simulink model "conveyor_belt_openloop"  (R2026a)
settings: Solver=ode4  StartTime=0  StopTime=20  FixedStep=0.01
PostLoadFcn:
  | mdlDir = fileparts(get_param('conveyor_belt_openloop', 'FileName'));
  | cadDir = fullfile(mdlDir, 'CAD');
  | addpath(cadDir);
  | prevDir = cd(cadDir);   % the copy in this folder wins over any other on the path
  | try
  |     convP = conveyor_belt_params();
  | catch paramsErr
  |     cd(prevDir); rethrow(paramsErr);
  | end
  | cd(prevDir);
  | missingFields = setdiff({'Ke', 'Tfric_Nm', 'bedFriction', 'beltDrag_N', 'beltTop_m', 'binFriction', 'contactOmega', 'contactZeta', 'controlPeriod_s', 'countsPerMotorRev', 'cycle_s', 'driverDrop_V', 'dropTimes_s', 'encWindow', 'frictionRate', 'g', 'gearEff', 'gearRatio', 'handOmega', 'handTime_s', 'itemFriction', 'itemMass_kg', 'itemSize_m', 'mmPerCount', 'motorR_ohm', 'rEff_m', 'restOffset_m', 'supplyV', 'vSlip', 'wSlip', 'xDrive_m', 'xDrop_m', 'xIdler_m', 'xReturn_m', 'zBinFloor_m', 'zCarry_m', 'zUnder_m', 'zWait_m'}, fieldnames(convP));
  | if ~isempty(missingFields)
  |     warning('Conveyor:params', '%s is older than this model (no %s). Replace it with the conveyor_belt_params.m that came with the model.', fullfile(cadDir, 'conveyor_belt_params.m'), strjoin(missingFields, ', '));
  | end
  | clear mdlDir cadDir prevDir missingFields
InitFcn:
  | mdlDir = fileparts(get_param('conveyor_belt_openloop', 'FileName'));
  | cadDir = fullfile(mdlDir, 'CAD');
  | addpath(cadDir);
  | prevDir = cd(cadDir);   % the copy in this folder wins over any other on the path
  | try
  |     convP = conveyor_belt_params();
  | catch paramsErr
  |     cd(prevDir); rethrow(paramsErr);
  | end
  | cd(prevDir);
  | missingFields = setdiff({'Ke', 'Tfric_Nm', 'bedFriction', 'beltDrag_N', 'beltTop_m', 'binFriction', 'contactOmega', 'contactZeta', 'controlPeriod_s', 'countsPerMotorRev', 'cycle_s', 'driverDrop_V', 'dropTimes_s', 'encWindow', 'frictionRate', 'g', 'gearEff', 'gearRatio', 'handOmega', 'handTime_s', 'itemFriction', 'itemMass_kg', 'itemSize_m', 'mmPerCount', 'motorR_ohm', 'rEff_m', 'restOffset_m', 'supplyV', 'vSlip', 'wSlip', 'xDrive_m', 'xDrop_m', 'xIdler_m', 'xReturn_m', 'zBinFloor_m', 'zCarry_m', 'zUnder_m', 'zWait_m'}, fieldnames(convP));
  | if isfield(convP, 'plaChain') && convP.plaChain ~= 0
  |     warning('Conveyor:belt', 'plaChain in conveyor_belt_params.m changed since this model was built: run build_conveyor_models so the 3-D parts match.');
  | end
  | if ~isempty(missingFields)
  |     error('Conveyor:params', '%s is older than this model (no %s). Replace it with the conveyor_belt_params.m that came with the model.', fullfile(cadDir, 'conveyor_belt_params.m'), strjoin(missingFields, ', '));
  | end
  | if ~strcmpi(pwd, mdlDir), cd(mdlDir); end   % STEP files are loaded as CAD/<part>.step
  | clear mdlDir cadDir prevDir missingFields
undefined symbols (not defined in the file or in its folder): X, Y, Z
libraries: sm_lib x73, nesl_utility x53, simulink x3, aerolibanimutils x1, slpidlib x1
(part 1 of 3)
settings Model: Creator=natha  LastModifiedBy=CadeP
settings SimscapeCC: SimscapeNominalValues="[{\"value\":\"1\",\"unit\":\"A\"},{\"value\":\"1\",\"unit\":\"bar\"},{\"value\":\"1\",\"unit\":\"cm^2\"},{\"value\":\"1\",\"unit\":\"cm^3/s\"},{\"value\":\"1\",\"unit\":\"kJ/kg\"},{\"value\":\"1\",\"unit\":\"kW\"},{\"value\":\"1\",\"unit\":\"l\"},{\"value\":\"1\",\"unit\":\"N\"},{\"value\":\"1\",\"unit\":\"N*m\"},{\"value\":\"1\",\"unit\":\"V\"}]"  SimscapeLogType=none  SimscapeLogDataHistory=5000.0

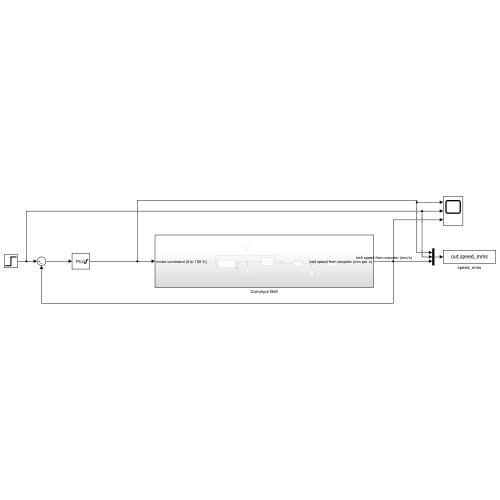
[thumbnail: Simulink's stored preview of the top-level diagram]
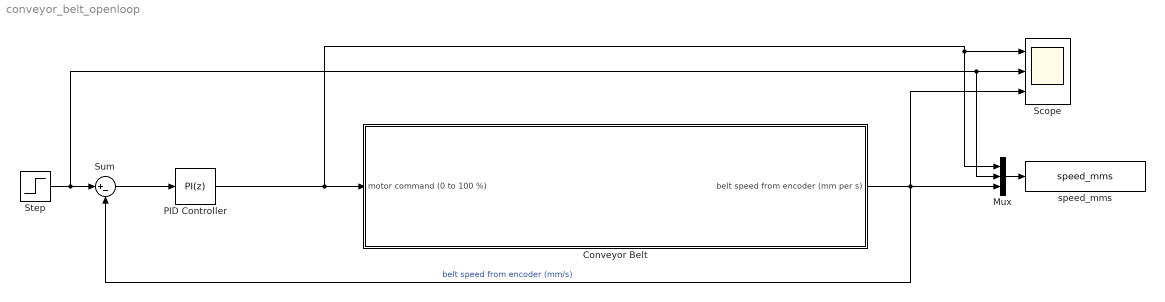
== system conveyor_belt_openloop ==
  Conveyor Belt : Subsystem
  Mux : Mux  Inputs=3
  PID Controller : slpidlib/PID Controller  Controller=PI  Form=Parallel  TimeDomain=Discrete-time  UseExternalTs=off  SampleTime=0.01  IntegratorMethod=Forward Euler  FilterMethod=Forward Euler  ControllerParametersSource=internal  P=0.0719  I=0.933  UseKiTs=off  D=0  UseExternalDerivativeSource=off  N=100  UseFilter=on  TunerSelectOption=Transfer Function Based (PID Tuner App)  InitialConditionSource=internal  InitialConditionForIntegrator=40  InitialConditionForFilter=0  DifferentiatorICPrevScaledInput=0  ExternalReset=none  TrackingMode=off  Kt=1  LimitOutput=on  SatLimitsSource=internal  UpperSaturationLimit=100  LowerSaturationLimit=25  LinearizeAsGain=on  AntiWindupMode=clamping  Kb=1  LimitIntegrator=off  UpperIntegratorSaturationLimit=inf  LowerIntegratorSaturationLimit=-inf  POutMin=[]  POutMax=[]  IOutMin=[]  IOutMax=[]  DOutMin=[]  DOutMax=[]  NOutMin=[]  NOutMax=[]  SumOutMin=[]  SumOutMax=[]  SaturationOutMin=[]  SaturationOutMax=[]  PParamMin=[]  PParamMax=[]  IParamMin=[]  IParamMax=[]  DParamMin=[]  DParamMax=[]  NParamMin=[]  NParamMax=[]  KbParamMin=[]  KbParamMax=[]  KtParamMin=[]  KtParamMax=[]  KbOutMin=[]  KbOutMax=[]  KtOutMin=[]  KtOutMax=[]  IntegratorOutMin=[]  IntegratorOutMax=[]  FilterOutMin=[]  FilterOutMax=[]  SumI1OutMin=[]  SumI1OutMax=[]  SumI2OutMin=[]  SumI2OutMax=[]  SumI3OutMin=[]  SumI3OutMax=[]  SumI4OutMin=[]  SumI4OutMax=[]  SumDOutMin=[]  SumDOutMax=[]  DifferentiatorOutMin=[]  DifferentiatorOutMax=[]  FilterDiffOutCoefMin=[]  FilterDiffOutCoefMax=[]  ReciprocalOutMin=[]  ReciprocalOutMax=[]  SumDenOutMin=[]  SumDenOutMax=[]  SumNumOutMin=[]  SumNumOutMax=[]  DivideOutMin=[]  DivideOutMax=[]  UdiffTsProdOutMin=[]  UdiffTsProdOutMax=[]  NTsProdOutMin=[]  NTsProdOutMax=[]  UintegralTsProdOutMin=[]  UintegralTsProdOutMax=[]  UngainTsProdOutMin=[]  UngainTsProdOutMax=[]  ClampingZeroOutDataTypeStr=Inherit: Inherit via back propagation  ClampingZeroOutMin=[]  ClampingZeroOutMax=[]  FilterDenConstantOutDataTypeStr=Inherit: Inherit via back propagation  FilterDenConstantOutMin=[]  FilterDenConstantOutMax=[]  PCopyOutDataTypeStr=Inherit: Inherit via back propagation  PCopyOutMin=[]  PCopyOutMax=[]  NCopyOutDataTypeStr=Inherit: Inherit via back propagation  NCopyOutMin=[]  NCopyOutMax=[]  IntegratorContinuousStateAttributes=''  IntegratorStateMustResolveToSignalObject=off  IntegratorRTWStateStorageClass=Auto  FilterContinuousStateAttributes=''  FilterStateMustResolveToSignalObject=off  FilterRTWStateStorageClass=Auto  ParallelPVariant=InternalParameters  IdealPVariant=Disabled  IVariant=InternalParameters  DVariant=Disabled  IntegratorVariant=Discrete  SatVariant=Enabled  AWVariant=DiscClampingParallel  PCopyVariant=Disabled  TRVariant=Disabled  FdbkBlocksVariant=Forward  IdealPFdbkVariant=Disabled  SatFdbkVariant=Disabled  DerivativeFilterVariant=Disabled  NVariant=Disabled  NCopyVariant=Disabled_SignalSpec  FilterICVariant=Disabled  IntegratorICVariant=InternalICs  ExternalResetVariant=Disabled  TRSumVariant=Passthrough  SumFdbkVariant=Disabled  SumVariant=Sum_PI  TsampFilterVariant=InternalTs  TsampNgainVariant=Passthrough  TsampIntegralVariant=Disabled_SignalSpec  ExternalSaturationOutDataTypeStr=Inherit: Same as second input  DerivativeSourceVariant=Disabled  PreIntVariant=InternalPreInt
  Scope : Scope  NumInputPorts=3
      settings: Title=motor command (% duty)  ActiveDisplayYMinimum=-122.04016461700802  ActiveDisplayYMaximum=1098.3614815530725
  Step : Step  Time=5  InitialValue=330  FinalValue=430  SampleTime=0
  Sum : Sum  Inputs=|+-
  speed_mms : ToWorkspace  VariableName=speed_mms  SaveFormat=Timeseries  SampleTime=-1
  wires:
  Conveyor Belt/1(belt speed from encoder (mm per s)) -> Sum/2, Mux/3, Scope/3  "belt speed from encoder (mm/s)"
  Mux/1 -> speed_mms/1
  PID Controller/1 -> Mux/1, Scope/1, Conveyor Belt/1(motor command (0 to 100 %))
  Step/1 -> Mux/2, Scope/2, Sum/1
  Sum/1 -> PID Controller/1

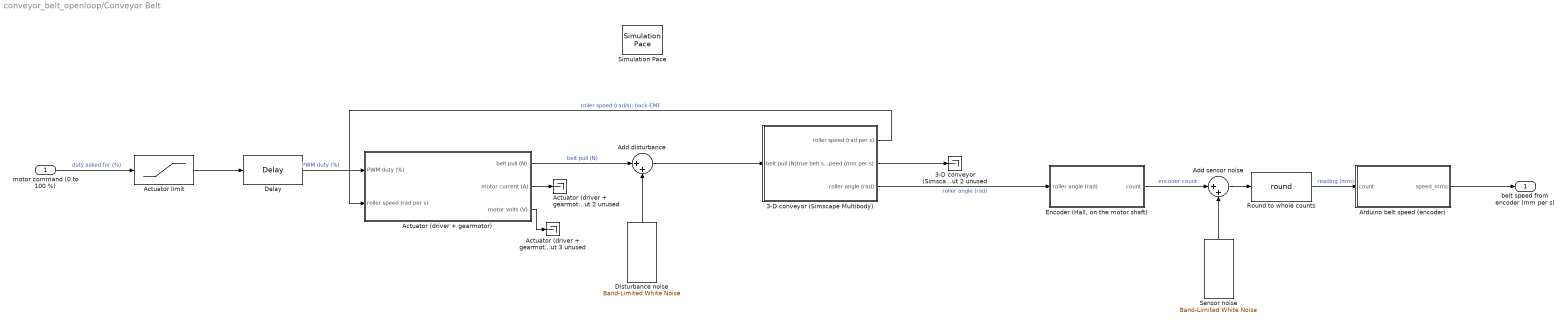
== system conveyor_belt_openloop/Conveyor Belt ==
  motor command (0 to 100 %) : Inport
  3-D conveyor (Simscape Multibody) : Subsystem
  3-D conveyor (Simscape Multibody) out 2 unused : Terminator
  Actuator (driver + gearmotor) : Subsystem
  Actuator (driver + gearmotor) out 2 unused : Terminator
  Actuator (driver + gearmotor) out 3 unused : Terminator
  Actuator limit : Saturate  UpperLimit=100  LowerLimit=0
  Add disturbance : Sum  Inputs=|++
  Add sensor noise : Sum  Inputs=|++
  Arduino belt speed (encoder) : MATLAB Function  TreatAsAtomicUnit=on
  Delay : TransportDelay  DelayTime=convP.delayBlock_s
  Disturbance noise : simulink/Sources/Band-Limited White Noise  Cov=convP.dragNoiseCov  Ts=convP.dragNoiseTs_s  seed=convP.noiseSeed + 1
  "Encoder (Hall, on the motor shaft)" : Subsystem
  Round to whole counts : Rounding  Operator=round
  Sensor noise : simulink/Sources/Band-Limited White Noise  Cov=0  Ts=0.01  seed=convP.noiseSeed
  Simulation Pace : aerolibanimutils/Simulation Pace  SimulationPace=1  SleepMode=Auto  OutputPaceError=off  SampleTime=-1
  belt speed from encoder (mm per s) : Outport
  wires:
  motor command (0 to 100 %)/1 -> Actuator limit/1  "duty asked for (%)"
  Actuator limit/1 -> Delay/1
  Delay/1 -> Actuator (driver + gearmotor)/1(PWM duty (%))  "PWM duty (%)"
  Actuator (driver + gearmotor)/1(belt pull (N)) -> Add disturbance/1  "belt pull (N)"
  Disturbance noise/1 -> Add disturbance/2
  Add disturbance/1 -> 3-D conveyor (Simscape Multibody)/1(belt pull (N))
  3-D conveyor (Simscape Multibody)/1(roller speed (rad per s)) -> Actuator (driver + gearmotor)/2(roller speed (rad per s))  "roller speed (rad/s): back-EMF"
  3-D conveyor (Simscape Multibody)/3(roller angle (rad)) -> "Encoder (Hall, on the motor shaft)"/1(roller angle (rad))  "roller angle (rad)"
  "Encoder (Hall, on the motor shaft)"/1(count) -> Add sensor noise/1  "encoder count"
  3-D conveyor (Simscape Multibody)/2(true belt speed (mm per s)) -> 3-D conveyor (Simscape Multibody) out 2 unused/1
  Actuator (driver + gearmotor)/2(motor current (A)) -> Actuator (driver + gearmotor) out 2 unused/1
  Actuator (driver + gearmotor)/3(motor volts (V)) -> Actuator (driver + gearmotor) out 3 unused/1
  Arduino belt speed (encoder)/1(speed_mms) -> belt speed from encoder (mm per s)/1
  Sensor noise/1 -> Add sensor noise/2
  Add sensor noise/1 -> Round to whole counts/1
  Round to whole counts/1 -> Arduino belt speed (encoder)/1(count)  "reading (mm)"

== system conveyor_belt_openloop/Conveyor Belt/3-D conveyor (Simscape Multibody) ==
  belt pull (N) : Inport
  Belt and item contact : MATLAB Function  TreatAsAtomicUnit=on
  Clock : Clock
  Drive roller : Subsystem
  Frame (fixed parts) : Subsystem
  Idler (follows the drive roller) : Subsystem
  Items : Subsystem
  Mechanism (gravity -Z) : sm_lib/Utilities/Mechanism Configuration  UniformGravity=Constant  GravityVector=[0 0 -9.80665]  GravityVectorUnits=m/s^2  LinearizationDelta=0.001  JointModeTransitionNonlinearIterations=2
  Net belt force : Sum  Inputs=|+-
  Solver : nesl_utility/Solver Configuration  PhysicalDomain=network_engine_domain  SubClassName=solver  LeftPortType=input  RightPortType=generic  Tones=[]  Harmonics=[]  SimulateNoise=off  Profile=off  UseLocalSampling=off  EnableSwitchedLinearOptims=on  FrequencyDomain=off  UseCCode=off  RelTol=0.001  AbsTol=0.001  MinStep=1e-09  ToWorkspace=off  RevertToSquareIcSolve=off  NumHomotopyIterations=100  PhasorMode=off  PhasorModeNumHarmonics=1  ConsistencySolver=NEWTON_XTOL_AFTER_FTOL  CanonicalOrdering=UNORDERED  OptimizeIntermediates=UNOPTIMIZED  IndexReductionMethod=DerivativeReplacement  DoDC=off  ResidualTolerance=1e-09  ConsistencyTolSource=GLOBAL  ConsistencyAbsTol=0.001  ConsistencyRelTol=0.001  ConsistencyTolFactor=0.001  UseLocalSolver=off  LocalSolverChoice=NE_BACKWARD_EULER_ADVANCER  ResolveIndetEquations=on  FunctionEvalNumThread=1  LocalSolverSampleTime=0.001  DoFixedCost=off  MaxNonlinIter=3  MaxModeIter=2  ComputeImpulses=off  ImpulseIterations=2  LinearAlgebra=auto  LinearAlgebraNumThread=0  EquationFormulation=NE_TIME_EF  DelaysMemoryBudget=1024  AutomaticFiltering=on  FilteringTimeConstant=0.001  PartitionStorageMethod=AS_NEEDED  PartitionMemoryBudget=1024  PartitionMethod=ROBUST  MultibodyUseLocalSolver=off  MultibodyLocalSolverChoice=ODE1  MultibodyLocalSolverSampleTime=0.001
  World : sm_lib/Frames and Transforms/World Frame
  belt speed (m per s) : Gain  Gain=convP.rEff_m
  times roller radius : Gain  Gain=convP.rEff_m
  to mm per s : Gain  Gain=1000
  roller speed (rad per s) : Outport
  true belt speed (mm per s) : Outport  Port=2
  roller angle (rad) : Outport  Port=3
  wires:
  belt pull (N)/1 -> Net belt force/1
  Belt and item contact/3(Fload) -> Net belt force/2  "load from items + bed drag (N)"
  Net belt force/1 -> times roller radius/1
  times roller radius/1 -> Drive roller/1(torque (N m))  "torque (N m)"
  Drive roller/1(angle (rad)) -> Idler (follows the drive roller)/1(drive roller angle (rad)), roller angle (rad)/1
  Drive roller/2(speed (rad per s)) -> belt speed (m per s)/1, roller speed (rad per s)/1
  belt speed (m per s)/1 -> Belt and item contact/5(vBelt), to mm per s/1
  to mm per s/1 -> true belt speed (mm per s)/1
  Clock/1 -> Belt and item contact/6(tNow)
  Items/1(x from drop point (m)) -> Belt and item contact/1(px)
  Items/2(z from drop point (m)) -> Belt and item contact/2(pz)
  Items/3(vx (m per s)) -> Belt and item contact/3(vx)
  Items/4(vz (m per s)) -> Belt and item contact/4(vz)
  Belt and item contact/1(Fx) -> Items/1(Fx (N))
  Belt and item contact/2(Fz) -> Items/2(Fz (N))
  connections:
  Solver/RConn1 -- World/RConn1 -- Items/LConn1 -- Drive roller/LConn1 -- Idler (follows the drive roller)/LConn1 -- Frame (fixed parts)/LConn1 -- Mechanism (gravity -Z)/RConn1

== system conveyor_belt_openloop/Conveyor Belt/Actuator (driver + gearmotor) ==
  PWM duty (%) : Inport
  roller speed (rad per s) : Inport  Port=2
  DC motor and gearbox : MATLAB Function  TreatAsAtomicUnit=on
  duty to volts : Gain  Gain=convP.supplyV/100
  belt pull (N) : Outport
  motor current (A) : Outport  Port=2
  motor volts (V) : Outport  Port=3
  wires:
  PWM duty (%)/1 -> duty to volts/1
  duty to volts/1 -> DC motor and gearbox/1(Vcmd)
  roller speed (rad per s)/1 -> DC motor and gearbox/2(wRoller)
  DC motor and gearbox/1(Fpull) -> belt pull (N)/1
  DC motor and gearbox/2(current) -> motor current (A)/1
  DC motor and gearbox/3(Vmotor) -> motor volts (V)/1

== system conveyor_belt_openloop/Conveyor Belt/Encoder (Hall, on the motor shaft) ==
  roller angle (rad) : Inport
  Edge jitter : simulink/Sources/Band-Limited White Noise  Cov=convP.encNoiseCov  Ts=convP.controlPeriod_s  seed=convP.noiseSeed + 2
  Hall encoder count : MATLAB Function  TreatAsAtomicUnit=on
  Read the count every 10 ms : ZeroOrderHold  SampleTime=convP.controlPeriod_s
  count : Outport
  wires:
  roller angle (rad)/1 -> Read the count every 10 ms/1
  Read the count every 10 ms/1 -> Hall encoder count/1(angle_rad)
  Edge jitter/1 -> Hall encoder count/2(jitter_counts)
  Hall encoder count/1(count) -> count/1

== system conveyor_belt_openloop/Conveyor Belt/3-D conveyor (Simscape Multibody)/Drive roller ==
  torque (N m) : Inport
  Drive axis : sm_lib/Frames and Transforms/Rigid Transform  RotationMethod=StandardAxis  FollAlignAxisA=+X  BaseAlignAxisA=+Y  FollAlignAxisB=+Y  BaseAlignAxisB=+Z  RotationStandardAxis=+X  RotationAngle=-90  RotationAngleUnits=deg  RotationArbitraryAxis=[0 0 1]  RotationSequenceAxes=FollowerAxes  RotationSequence=XYX  RotationSequenceAngles=[0 0 0]  RotationSequenceAnglesUnits=deg  RotationMatrix=[1 0 0;0 1 0;0 0 1]  Quaternion=[1 0 0 0]  TranslationMethod=Cartesian  TranslationCartesianOffset=[convP.xDrive_m 0 convP.zAxis_m]  TranslationCartesianOffsetUnits=m  TranslationStandardAxis=+Z  TranslationStandardOffset=0  TranslationStandardOffsetUnits=m  TranslationROffset=0  TranslationROffsetUnits=m  TranslationThetaOffset=0  TranslationThetaOffsetUnits=deg  TranslationZOffset=0  TranslationZOffsetUnits=m
  Drive roller bearings : sm_lib/Joints/Revolute Joint  JointMode=Normal  CompositeWrenchDir=FollowerOnBase  CompositeWrenchFrame=BaseFrame  SenseConstraintForce=off  SenseConstraintTorque=off  SenseTotalForce=off  SenseTotalTorque=off  PositionTargetSpecify=off  PositionTargetPriority=High  PositionTargetValue=0  PositionTargetValueUnits=deg  VelocityTargetSpecify=off  VelocityTargetPriority=High  VelocityTargetValue=0  VelocityTargetValueUnits=deg/s  EquilibriumPosition=0  EquilibriumPositionUnits=deg  SpringStiffness=0  SpringStiffnessUnits=N*m/deg  DampingCoefficient=0  DampingCoefficientUnits=N*m/(deg/s)  LowerLimitSpecify=off  LowerLimitBound=-90  LowerLimitBoundUnits=deg  LowerLimitStiffness=1e4  LowerLimitStiffnessUnits=N*m/deg  LowerLimitDamping=10  LowerLimitDampingUnits=N*m/(deg/s)  LowerLimitTransitionRegionWidth=0.1  LowerLimitTransitionRegionWidthUnits=deg  UpperLimitSpecify=off  UpperLimitBound=90  UpperLimitBoundUnits=deg  UpperLimitStiffness=1e4  UpperLimitStiffnessUnits=N*m/deg  UpperLimitDamping=10  UpperLimitDampingUnits=N*m/(deg/s)  UpperLimitTransitionRegionWidth=0.1  UpperLimitTransitionRegionWidthUnits=deg  TorqueActuationMode=InputTorque  MotionActuationMode=ComputedMotion  SensePosition=on  SenseVelocity=on  SenseAcceleration=off  SenseTorqueForce=off  SenseLowerLimitTorqueForce=off  SenseUpperLimitTorqueForce=off
  Motor rotor (reflected inertia) : sm_lib/Body Elements/Inertia  InertiaType=Custom  Mass=0.01  MassUnits=kg  CenterOfMass=[0 0 0]  CenterOfMassUnits=m  MomentsOfInertia=[1 1 1]*convP.J_drive  MomentsOfInertiaUnits=kg*m^2  ProductsOfInertia=[0 0 0]  ProductsOfInertiaUnits=kg*m^2  GraphicType=Marker  MarkerShape=Inertia  MarkerSize=20  GraphicVisPropType=SimpleVisualProperties  GraphicDiffuseColor=[0.5 0.5 0.5]  GraphicOpacity=1  GraphicSpecularColor=[0.5 0.5 0.5 1.0]  GraphicAmbientColor=[0.15 0.15 0.15 1.0]  GraphicEmissiveColor=[0.0 0.0 0.0 1.0]  GraphicShininess=75
  Other half faces the other way : sm_lib/Frames and Transforms/Rigid Transform  RotationMethod=StandardAxis  FollAlignAxisA=+X  BaseAlignAxisA=+Y  FollAlignAxisB=+Y  BaseAlignAxisB=+Z  RotationStandardAxis=+X  RotationAngle=180  RotationAngleUnits=deg  RotationArbitraryAxis=[0 0 1]  RotationSequenceAxes=FollowerAxes  RotationSequence=XYX  RotationSequenceAngles=[0 0 0]  RotationSequenceAnglesUnits=deg  RotationMatrix=[1 0 0;0 1 0;0 0 1]  Quaternion=[1 0 0 0]  TranslationMethod=None  TranslationCartesianOffset=[0 0 0]  TranslationCartesianOffsetUnits=m  TranslationStandardAxis=+Z  TranslationStandardOffset=0  TranslationStandardOffsetUnits=m  TranslationROffset=0  TranslationROffsetUnits=m  TranslationThetaOffset=0  TranslationThetaOffsetUnits=deg  TranslationZOffset=0  TranslationZOffsetUnits=m
  Roller half (drive end) : sm_lib/Body Elements/File Solid  ExtGeomFileName=CAD/roller_half_drive.step  UnitType=FromFile  ExtGeomFileUnits=m  StepReaderType=HEX  ExportConvexHullGeometry=off  InertiaType=CalculateFromGeometry  BasedOnType=Density  Density=convP.printDensity_kgm3  DensityUnits=kg/m^3  Mass=1  MassUnits=kg  CenterOfMass=[0 0 0]  CenterOfMassUnits=m  MomentsOfInertia=[1 1 1]  MomentsOfInertiaUnits=kg*m^2  ProductsOfInertia=[0 0 0]  ProductsOfInertiaUnits=kg*m^2  GraphicType=FromGeometry  MarkerShape=Sphere  MarkerSize=10  GraphicVisPropType=SimpleVisualProperties  GraphicDiffuseColor=[0.92 0.92 0.92]  GraphicOpacity=1  GraphicSpecularColor=[0.5 0.5 0.5 1.0]  GraphicAmbientColor=[0.15 0.15 0.15 1.0]  GraphicEmissiveColor=[0.0 0.0 0.0 1.0]  GraphicShininess=75  DoExposeReferenceFrame=on  SerializedFrames=<Frames/>
  Roller half (plain end) : sm_lib/Body Elements/File Solid  ExtGeomFileName=CAD/roller_half_plain.step  UnitType=FromFile  ExtGeomFileUnits=m  StepReaderType=HEX  ExportConvexHullGeometry=off  InertiaType=CalculateFromGeometry  BasedOnType=Density  Density=convP.printDensity_kgm3  DensityUnits=kg/m^3  Mass=1  MassUnits=kg  CenterOfMass=[0 0 0]  CenterOfMassUnits=m  MomentsOfInertia=[1 1 1]  MomentsOfInertiaUnits=kg*m^2  ProductsOfInertia=[0 0 0]  ProductsOfInertiaUnits=kg*m^2  GraphicType=FromGeometry  MarkerShape=Sphere  MarkerSize=10  GraphicVisPropType=SimpleVisualProperties  GraphicDiffuseColor=[0.92 0.92 0.92]  GraphicOpacity=1  GraphicSpecularColor=[0.5 0.5 0.5 1.0]  GraphicAmbientColor=[0.15 0.15 0.15 1.0]  GraphicEmissiveColor=[0.0 0.0 0.0 1.0]  GraphicShininess=75  DoExposeReferenceFrame=on  SerializedFrames=<Frames/>
  angle out : nesl_utility/PS-Simulink Converter  PhysicalDomain=network_engine_domain  SubClassName=ps_output  LeftPortType=input  RightPortType=output  PseudoPeriodic=off  Frequencies=[]  VectorFormat=inherit  Unit=rad  AffineConversion=off
  speed out : nesl_utility/PS-Simulink Converter  PhysicalDomain=network_engine_domain  SubClassName=ps_output  LeftPortType=input  RightPortType=output  PseudoPeriodic=off  Frequencies=[]  VectorFormat=inherit  Unit=rad/s  AffineConversion=off
  torque to physical : nesl_utility/Simulink-PS Converter  PhysicalDomain=network_engine_domain  SubClassName=ps_input  LeftPortType=input  RightPortType=output  PseudoPeriodic=off  Frequencies=[]  NoiseDistribution=none  NoiseParameters=[]  Unit=N*m  AffineConversion=off  FilteringAndDerivatives=provide  SimscapeFilterOrder=1  InputFilterTimeConstant=0.001  UdotUserProvided=0
  W : PMIOPort  Side=Left
  angle (rad) : Outport
  speed (rad per s) : Outport  Port=2
  wires:
  torque (N m)/1 -> torque to physical/1
  angle out/1 -> angle (rad)/1
  speed out/1 -> speed (rad per s)/1
  connections:
  W/RConn1 -- Drive axis/LConn1
  Drive axis/RConn1 -- Drive roller bearings/LConn1
  torque to physical/RConn1 -- Drive roller bearings/LConn2
  Roller half (drive end)/RConn1 -- Drive roller bearings/RConn1 -- Other half faces the other way/LConn1 -- Motor rotor (reflected inertia)/RConn1
  Other half faces the other way/RConn1 -- Roller half (plain end)/RConn1
  Drive roller bearings/RConn2 -- angle out/LConn1
  Drive roller bearings/RConn3 -- speed out/LConn1

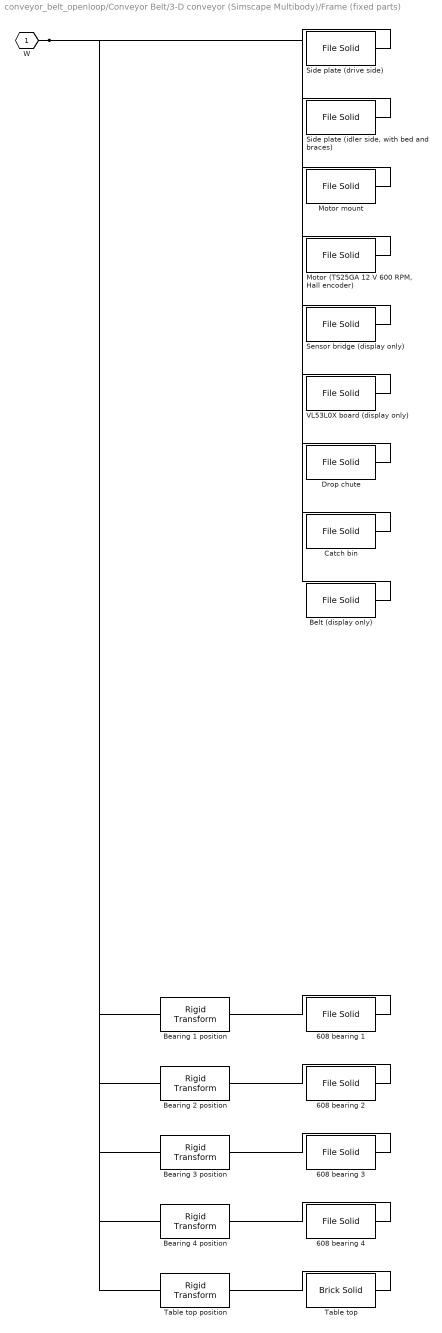
== system conveyor_belt_openloop/Conveyor Belt/3-D conveyor (Simscape Multibody)/Frame (fixed parts) ==
  608 bearing {1..4} (4 alike) : sm_lib/Body Elements/File Solid  ExtGeomFileName=CAD/bearing_608.step  UnitType=FromFile  ExtGeomFileUnits=m  StepReaderType=HEX  ExportConvexHullGeometry=off  InertiaType=CalculateFromGeometry  BasedOnType=Density  Density=convP.printDensity_kgm3  DensityUnits=kg/m^3  Mass=1  MassUnits=kg  CenterOfMass=[0 0 0]  CenterOfMassUnits=m  MomentsOfInertia=[1 1 1]  MomentsOfInertiaUnits=kg*m^2  ProductsOfInertia=[0 0 0]  ProductsOfInertiaUnits=kg*m^2  GraphicType=FromGeometry  MarkerShape=Sphere  MarkerSize=10  GraphicVisPropType=SimpleVisualProperties  GraphicDiffuseColor=[0.6 0.6 0.65]  GraphicOpacity=1  GraphicSpecularColor=[0.5 0.5 0.5 1.0]  GraphicAmbientColor=[0.15 0.15 0.15 1.0]  GraphicEmissiveColor=[0.0 0.0 0.0 1.0]  GraphicShininess=75  DoExposeReferenceFrame=on  SerializedFrames=<Frames/>
  Bearing 1 position : sm_lib/Frames and Transforms/Rigid Transform  RotationMethod=StandardAxis  FollAlignAxisA=+X  BaseAlignAxisA=+Y  FollAlignAxisB=+Y  BaseAlignAxisB=+Z  RotationStandardAxis=+X  RotationAngle=-90  RotationAngleUnits=deg  RotationArbitraryAxis=[0 0 1]  RotationSequenceAxes=FollowerAxes  RotationSequence=XYX  RotationSequenceAngles=[0 0 0]  RotationSequenceAnglesUnits=deg  RotationMatrix=[1 0 0;0 1 0;0 0 1]  Quaternion=[1 0 0 0]  TranslationMethod=Cartesian  TranslationCartesianOffset=[convP.xDrive_m convP.bearingY_m(1) convP.zAxis_m]  TranslationCartesianOffsetUnits=m  TranslationStandardAxis=+Z  TranslationStandardOffset=0  TranslationStandardOffsetUnits=m  TranslationROffset=0  TranslationROffsetUnits=m  TranslationThetaOffset=0  TranslationThetaOffsetUnits=deg  TranslationZOffset=0  TranslationZOffsetUnits=m
  Bearing 2 position : sm_lib/Frames and Transforms/Rigid Transform  RotationMethod=StandardAxis  FollAlignAxisA=+X  BaseAlignAxisA=+Y  FollAlignAxisB=+Y  BaseAlignAxisB=+Z  RotationStandardAxis=+X  RotationAngle=-90  RotationAngleUnits=deg  RotationArbitraryAxis=[0 0 1]  RotationSequenceAxes=FollowerAxes  RotationSequence=XYX  RotationSequenceAngles=[0 0 0]  RotationSequenceAnglesUnits=deg  RotationMatrix=[1 0 0;0 1 0;0 0 1]  Quaternion=[1 0 0 0]  TranslationMethod=Cartesian  TranslationCartesianOffset=[convP.xDrive_m convP.bearingY_m(2) convP.zAxis_m]  TranslationCartesianOffsetUnits=m  TranslationStandardAxis=+Z  TranslationStandardOffset=0  TranslationStandardOffsetUnits=m  TranslationROffset=0  TranslationROffsetUnits=m  TranslationThetaOffset=0  TranslationThetaOffsetUnits=deg  TranslationZOffset=0  TranslationZOffsetUnits=m
  Bearing 3 position : sm_lib/Frames and Transforms/Rigid Transform  RotationMethod=StandardAxis  FollAlignAxisA=+X  BaseAlignAxisA=+Y  FollAlignAxisB=+Y  BaseAlignAxisB=+Z  RotationStandardAxis=+X  RotationAngle=-90  RotationAngleUnits=deg  RotationArbitraryAxis=[0 0 1]  RotationSequenceAxes=FollowerAxes  RotationSequence=XYX  RotationSequenceAngles=[0 0 0]  RotationSequenceAnglesUnits=deg  RotationMatrix=[1 0 0;0 1 0;0 0 1]  Quaternion=[1 0 0 0]  TranslationMethod=Cartesian  TranslationCartesianOffset=[convP.xIdler_m convP.bearingY_m(1) convP.zAxis_m]  TranslationCartesianOffsetUnits=m  TranslationStandardAxis=+Z  TranslationStandardOffset=0  TranslationStandardOffsetUnits=m  TranslationROffset=0  TranslationROffsetUnits=m  TranslationThetaOffset=0  TranslationThetaOffsetUnits=deg  TranslationZOffset=0  TranslationZOffsetUnits=m
  Bearing 4 position : sm_lib/Frames and Transforms/Rigid Transform  RotationMethod=StandardAxis  FollAlignAxisA=+X  BaseAlignAxisA=+Y  FollAlignAxisB=+Y  BaseAlignAxisB=+Z  RotationStandardAxis=+X  RotationAngle=-90  RotationAngleUnits=deg  RotationArbitraryAxis=[0 0 1]  RotationSequenceAxes=FollowerAxes  RotationSequence=XYX  RotationSequenceAngles=[0 0 0]  RotationSequenceAnglesUnits=deg  RotationMatrix=[1 0 0;0 1 0;0 0 1]  Quaternion=[1 0 0 0]  TranslationMethod=Cartesian  TranslationCartesianOffset=[convP.xIdler_m convP.bearingY_m(2) convP.zAxis_m]  TranslationCartesianOffsetUnits=m  TranslationStandardAxis=+Z  TranslationStandardOffset=0  TranslationStandardOffsetUnits=m  TranslationROffset=0  TranslationROffsetUnits=m  TranslationThetaOffset=0  TranslationThetaOffsetUnits=deg  TranslationZOffset=0  TranslationZOffsetUnits=m
  Belt (display only) : sm_lib/Body Elements/File Solid  ExtGeomFileName=CAD/belt_installed_display.step  UnitType=FromFile  ExtGeomFileUnits=m  StepReaderType=HEX  ExportConvexHullGeometry=off  InertiaType=CalculateFromGeometry  BasedOnType=Density  Density=convP.printDensity_kgm3  DensityUnits=kg/m^3  Mass=1  MassUnits=kg  CenterOfMass=[0 0 0]  CenterOfMassUnits=m  MomentsOfInertia=[1 1 1]  MomentsOfInertiaUnits=kg*m^2  ProductsOfInertia=[0 0 0]  ProductsOfInertiaUnits=kg*m^2  GraphicType=FromGeometry  MarkerShape=Sphere  MarkerSize=10  GraphicVisPropType=SimpleVisualProperties  GraphicDiffuseColor=[0.1 0.1 0.1]  GraphicOpacity=1  GraphicSpecularColor=[0.5 0.5 0.5 1.0]  GraphicAmbientColor=[0.15 0.15 0.15 1.0]  GraphicEmissiveColor=[0.0 0.0 0.0 1.0]  GraphicShininess=75  DoExposeReferenceFrame=on  SerializedFrames=<Frames/>
  Catch bin : sm_lib/Body Elements/File Solid  ExtGeomFileName=CAD/catch_bin.step  UnitType=FromFile  ExtGeomFileUnits=m  StepReaderType=HEX  ExportConvexHullGeometry=off  InertiaType=CalculateFromGeometry  BasedOnType=Density  Density=convP.printDensity_kgm3  DensityUnits=kg/m^3  Mass=1  MassUnits=kg  CenterOfMass=[0 0 0]  CenterOfMassUnits=m  MomentsOfInertia=[1 1 1]  MomentsOfInertiaUnits=kg*m^2  ProductsOfInertia=[0 0 0]  ProductsOfInertiaUnits=kg*m^2  GraphicType=FromGeometry  MarkerShape=Sphere  MarkerSize=10  GraphicVisPropType=SimpleVisualProperties  GraphicDiffuseColor=[0.45 0.45 0.45]  GraphicOpacity=1  GraphicSpecularColor=[0.5 0.5 0.5 1.0]  GraphicAmbientColor=[0.15 0.15 0.15 1.0]  GraphicEmissiveColor=[0.0 0.0 0.0 1.0]  GraphicShininess=75  DoExposeReferenceFrame=on  SerializedFrames=<Frames/>
  Drop chute : sm_lib/Body Elements/File Solid  ExtGeomFileName=CAD/drop_chute.step  UnitType=FromFile  ExtGeomFileUnits=m  StepReaderType=HEX  ExportConvexHullGeometry=off  InertiaType=CalculateFromGeometry  BasedOnType=Density  Density=convP.printDensity_kgm3  DensityUnits=kg/m^3  Mass=1  MassUnits=kg  CenterOfMass=[0 0 0]  CenterOfMassUnits=m  MomentsOfInertia=[1 1 1]  MomentsOfInertiaUnits=kg*m^2  ProductsOfInertia=[0 0 0]  ProductsOfInertiaUnits=kg*m^2  GraphicType=FromGeometry  MarkerShape=Sphere  MarkerSize=10  GraphicVisPropType=SimpleVisualProperties  GraphicDiffuseColor=[0.15 0.65 0.35]  GraphicOpacity=1  GraphicSpecularColor=[0.5 0.5 0.5 1.0]  GraphicAmbientColor=[0.15 0.15 0.15 1.0]  GraphicEmissiveColor=[0.0 0.0 0.0 1.0]  GraphicShininess=75  DoExposeReferenceFrame=on  SerializedFrames=<Frames/>
  "Motor (TS25GA 12 V 600 RPM, Hall encoder)" : sm_lib/Body Elements/File Solid  ExtGeomFileName=CAD/motor_ts25ga_12v.step  UnitType=FromFile  ExtGeomFileUnits=m  StepReaderType=HEX  ExportConvexHullGeometry=off  InertiaType=CalculateFromGeometry  BasedOnType=Density  Density=convP.printDensity_kgm3  DensityUnits=kg/m^3  Mass=1  MassUnits=kg  CenterOfMass=[0 0 0]  CenterOfMassUnits=m  MomentsOfInertia=[1 1 1]  MomentsOfInertiaUnits=kg*m^2  ProductsOfInertia=[0 0 0]  ProductsOfInertiaUnits=kg*m^2  GraphicType=FromGeometry  MarkerShape=Sphere  MarkerSize=10  GraphicVisPropType=SimpleVisualProperties  GraphicDiffuseColor=[0.8 0.8 0.85]  GraphicOpacity=1  GraphicSpecularColor=[0.5 0.5 0.5 1.0]  GraphicAmbientColor=[0.15 0.15 0.15 1.0]  GraphicEmissiveColor=[0.0 0.0 0.0 1.0]  GraphicShininess=75  DoExposeReferenceFrame=on  SerializedFrames=<Frames/>
  Motor mount : sm_lib/Body Elements/File Solid  ExtGeomFileName=CAD/motor_mount.step  UnitType=FromFile  ExtGeomFileUnits=m  StepReaderType=HEX  ExportConvexHullGeometry=off  InertiaType=CalculateFromGeometry  BasedOnType=Density  Density=convP.printDensity_kgm3  DensityUnits=kg/m^3  Mass=1  MassUnits=kg  CenterOfMass=[0 0 0]  CenterOfMassUnits=m  MomentsOfInertia=[1 1 1]  MomentsOfInertiaUnits=kg*m^2  ProductsOfInertia=[0 0 0]  ProductsOfInertiaUnits=kg*m^2  GraphicType=FromGeometry  MarkerShape=Sphere  MarkerSize=10  GraphicVisPropType=SimpleVisualProperties  GraphicDiffuseColor=[0.25 0.75 0.85]  GraphicOpacity=1  GraphicSpecularColor=[0.5 0.5 0.5 1.0]  GraphicAmbientColor=[0.15 0.15 0.15 1.0]  GraphicEmissiveColor=[0.0 0.0 0.0 1.0]  GraphicShininess=75  DoExposeReferenceFrame=on  SerializedFrames=<Frames/>
  Sensor bridge (display only) : sm_lib/Body Elements/File Solid  ExtGeomFileName=CAD/sensor_bridge.step  UnitType=FromFile  ExtGeomFileUnits=m  StepReaderType=HEX  ExportConvexHullGeometry=off  InertiaType=CalculateFromGeometry  BasedOnType=Density  Density=convP.printDensity_kgm3  DensityUnits=kg/m^3  Mass=1  MassUnits=kg  CenterOfMass=[0 0 0]  CenterOfMassUnits=m  MomentsOfInertia=[1 1 1]  MomentsOfInertiaUnits=kg*m^2  ProductsOfInertia=[0 0 0]  ProductsOfInertiaUnits=kg*m^2  GraphicType=FromGeometry  MarkerShape=Sphere  MarkerSize=10  GraphicVisPropType=SimpleVisualProperties  GraphicDiffuseColor=[0.15 0.65 0.35]  GraphicOpacity=1  GraphicSpecularColor=[0.5 0.5 0.5 1.0]  GraphicAmbientColor=[0.15 0.15 0.15 1.0]  GraphicEmissiveColor=[0.0 0.0 0.0 1.0]  GraphicShininess=75  DoExposeReferenceFrame=on  SerializedFrames=<Frames/>
  Side plate (drive side) : sm_lib/Body Elements/File Solid  ExtGeomFileName=CAD/side_plate_drive.step  UnitType=FromFile  ExtGeomFileUnits=m  StepReaderType=HEX  ExportConvexHullGeometry=off  InertiaType=CalculateFromGeometry  BasedOnType=Density  Density=convP.printDensity_kgm3  DensityUnits=kg/m^3  Mass=1  MassUnits=kg  CenterOfMass=[0 0 0]  CenterOfMassUnits=m  MomentsOfInertia=[1 1 1]  MomentsOfInertiaUnits=kg*m^2  ProductsOfInertia=[0 0 0]  ProductsOfInertiaUnits=kg*m^2  GraphicType=FromGeometry  MarkerShape=Sphere  MarkerSize=10  GraphicVisPropType=SimpleVisualProperties  GraphicDiffuseColor=[0.25 0.45 0.85]  GraphicOpacity=1  GraphicSpecularColor=[0.5 0.5 0.5 1.0]  GraphicAmbientColor=[0.15 0.15 0.15 1.0]  GraphicEmissiveColor=[0.0 0.0 0.0 1.0]  GraphicShininess=75  DoExposeReferenceFrame=on  SerializedFrames=<Frames/>
  "Side plate (idler side, with bed and braces)" : sm_lib/Body Elements/File Solid  ExtGeomFileName=CAD/side_plate_idler.step  UnitType=FromFile  ExtGeomFileUnits=m  StepReaderType=HEX  ExportConvexHullGeometry=off  InertiaType=CalculateFromGeometry  BasedOnType=Density  Density=convP.printDensity_kgm3  DensityUnits=kg/m^3  Mass=1  MassUnits=kg  CenterOfMass=[0 0 0]  CenterOfMassUnits=m  MomentsOfInertia=[1 1 1]  MomentsOfInertiaUnits=kg*m^2  ProductsOfInertia=[0 0 0]  ProductsOfInertiaUnits=kg*m^2  GraphicType=FromGeometry  MarkerShape=Sphere  MarkerSize=10  GraphicVisPropType=SimpleVisualProperties  GraphicDiffuseColor=[0.25 0.45 0.85]  GraphicOpacity=1  GraphicSpecularColor=[0.5 0.5 0.5 1.0]  GraphicAmbientColor=[0.15 0.15 0.15 1.0]  GraphicEmissiveColor=[0.0 0.0 0.0 1.0]  GraphicShininess=75  DoExposeReferenceFrame=on  SerializedFrames=<Frames/>
  Table top : sm_lib/Body Elements/Brick Solid  BrickDimensions=convP.tableSize_m  BrickDimensionsUnits=m  ExportEntireGeometry=off  InertiaType=CalculateFromGeometry  BasedOnType=Density  Density=700  DensityUnits=kg/m^3  Mass=1  MassUnits=kg  CenterOfMass=[0 0 0]  CenterOfMassUnits=m  MomentsOfInertia=[1 1 1]  MomentsOfInertiaUnits=kg*m^2  ProductsOfInertia=[0 0 0]  ProductsOfInertiaUnits=kg*m^2  GraphicType=FromGeometry  MarkerShape=Sphere  MarkerSize=10  GraphicVisPropType=SimpleVisualProperties  GraphicDiffuseColor=[0.80 0.68 0.50]  GraphicOpacity=1  GraphicSpecularColor=[0.5 0.5 0.5 1.0]  GraphicAmbientColor=[0.15 0.15 0.15 1.0]  GraphicEmissiveColor=[0.0 0.0 0.0 1.0]  GraphicShininess=75  DoExposeReferenceFrame=on  SerializedFrames=<Frames/>
  Table top position : sm_lib/Frames and Transforms/Rigid Transform  RotationMethod=None  FollAlignAxisA=+X  BaseAlignAxisA=+Y  FollAlignAxisB=+Y  BaseAlignAxisB=+Z  RotationStandardAxis=+Z  RotationAngle=0  RotationAngleUnits=deg  RotationArbitraryAxis=[0 0 1]  RotationSequenceAxes=FollowerAxes  RotationSequence=XYX  RotationSequenceAngles=[0 0 0]  RotationSequenceAnglesUnits=deg  RotationMatrix=[1 0 0;0 1 0;0 0 1]  Quaternion=[1 0 0 0]  TranslationMethod=Cartesian  TranslationCartesianOffset=convP.tableCentre_m  TranslationCartesianOffsetUnits=m  TranslationStandardAxis=+Z  TranslationStandardOffset=0  TranslationStandardOffsetUnits=m  TranslationROffset=0  TranslationROffsetUnits=m  TranslationThetaOffset=0  TranslationThetaOffsetUnits=deg  TranslationZOffset=0  TranslationZOffsetUnits=m
  VL53L0X board (display only) : sm_lib/Body Elements/File Solid  ExtGeomFileName=CAD/vl53l0x_board.step  UnitType=FromFile  ExtGeomFileUnits=m  StepReaderType=HEX  ExportConvexHullGeometry=off  InertiaType=CalculateFromGeometry  BasedOnType=Density  Density=convP.printDensity_kgm3  DensityUnits=kg/m^3  Mass=1  MassUnits=kg  CenterOfMass=[0 0 0]  CenterOfMassUnits=m  MomentsOfInertia=[1 1 1]  MomentsOfInertiaUnits=kg*m^2  ProductsOfInertia=[0 0 0]  ProductsOfInertiaUnits=kg*m^2  GraphicType=FromGeometry  MarkerShape=Sphere  MarkerSize=10  GraphicVisPropType=SimpleVisualProperties  GraphicDiffuseColor=[0.5 0.15 0.6]  GraphicOpacity=1  GraphicSpecularColor=[0.5 0.5 0.5 1.0]  GraphicAmbientColor=[0.15 0.15 0.15 1.0]  GraphicEmissiveColor=[0.0 0.0 0.0 1.0]  GraphicShininess=75  DoExposeReferenceFrame=on  SerializedFrames=<Frames/>
  W : PMIOPort  Side=Left
  connections:
  Side plate (drive side)/RConn1 -- W/RConn1 -- "Side plate (idler side, with bed and braces)"/RConn1 -- Motor mount/RConn1 -- "Motor (TS25GA 12 V 600 RPM, Hall encoder)"/RConn1 -- Sensor bridge (display only)/RConn1 -- VL53L0X board (display only)/RConn1 -- Drop chute/RConn1 -- Catch bin/RConn1 -- Belt (display only)/RConn1 -- Table top position/LConn1 -- Bearing 1 position/LConn1 -- Bearing 2 position/LConn1 -- Bearing 3 position/LConn1 -- Bearing 4 position/LConn1
  Table top position/RConn1 -- Table top/RConn1
  Bearing 1 position/RConn1 -- 608 bearing 1/RConn1
  Bearing 2 position/RConn1 -- 608 bearing 2/RConn1
  Bearing 3 position/RConn1 -- 608 bearing 3/RConn1
  Bearing 4 position/RConn1 -- 608 bearing 4/RConn1

== system conveyor_belt_openloop/Conveyor Belt/3-D conveyor (Simscape Multibody)/Idler (follows the drive roller) ==
  drive roller angle (rad) : Inport
  Idler roller angle : nesl_utility/Simulink-PS Converter  PhysicalDomain=network_engine_domain  SubClassName=ps_input  LeftPortType=input  RightPortType=output  PseudoPeriodic=off  Frequencies=[]  NoiseDistribution=none  NoiseParameters=[]  Unit=rad  AffineConversion=off  FilteringAndDerivatives=filter  SimscapeFilterOrder=2  InputFilterTimeConstant=0.03  UdotUserProvided=0
  Idler roller axis : sm_lib/Frames and Transforms/Rigid Transform  RotationMethod=StandardAxis  FollAlignAxisA=+X  BaseAlignAxisA=+Y  FollAlignAxisB=+Y  BaseAlignAxisB=+Z  RotationStandardAxis=+X  RotationAngle=-90  RotationAngleUnits=deg  RotationArbitraryAxis=[0 0 1]  RotationSequenceAxes=FollowerAxes  RotationSequence=XYX  RotationSequenceAngles=[0 0 0]  RotationSequenceAnglesUnits=deg  RotationMatrix=[1 0 0;0 1 0;0 0 1]  Quaternion=[1 0 0 0]  TranslationMethod=Cartesian  TranslationCartesianOffset=[convP.xIdler_m 0 convP.zAxis_m]  TranslationCartesianOffsetUnits=m  TranslationStandardAxis=+Z  TranslationStandardOffset=0  TranslationStandardOffsetUnits=m  TranslationROffset=0  TranslationROffsetUnits=m  TranslationThetaOffset=0  TranslationThetaOffsetUnits=deg  TranslationZOffset=0  TranslationZOffsetUnits=m
  Idler roller joint : sm_lib/Joints/Revolute Joint  JointMode=Normal  CompositeWrenchDir=FollowerOnBase  CompositeWrenchFrame=BaseFrame  SenseConstraintForce=off  SenseConstraintTorque=off  SenseTotalForce=off  SenseTotalTorque=off  PositionTargetSpecify=off  PositionTargetPriority=High  PositionTargetValue=0  PositionTargetValueUnits=deg  VelocityTargetSpecify=off  VelocityTargetPriority=High  VelocityTargetValue=0  VelocityTargetValueUnits=deg/s  EquilibriumPosition=0  EquilibriumPositionUnits=deg  SpringStiffness=0  SpringStiffnessUnits=N*m/deg  DampingCoefficient=0  DampingCoefficientUnits=N*m/(deg/s)  LowerLimitSpecify=off  LowerLimitBound=-90  LowerLimitBoundUnits=deg  LowerLimitStiffness=1e4  LowerLimitStiffnessUnits=N*m/deg  LowerLimitDamping=10  LowerLimitDampingUnits=N*m/(deg/s)  LowerLimitTransitionRegionWidth=0.1  LowerLimitTransitionRegionWidthUnits=deg  UpperLimitSpecify=off  UpperLimitBound=90  UpperLimitBoundUnits=deg  UpperLimitStiffness=1e4  UpperLimitStiffnessUnits=N*m/deg  UpperLimitDamping=10  UpperLimitDampingUnits=N*m/(deg/s)  UpperLimitTransitionRegionWidth=0.1  UpperLimitTransitionRegionWidthUnits=deg  TorqueActuationMode=ComputedTorque  MotionActuationMode=InputMotion  SensePosition=off  SenseVelocity=off  SenseAcceleration=off  SenseTorqueForce=off  SenseLowerLimitTorqueForce=off  SenseUpperLimitTorqueForce=off
  Idler roller other half faces the other way : sm_lib/Frames and Transforms/Rigid Transform  RotationMethod=StandardAxis  FollAlignAxisA=+X  BaseAlignAxisA=+Y  FollAlignAxisB=+Y  BaseAlignAxisB=+Z  RotationStandardAxis=+X  RotationAngle=180  RotationAngleUnits=deg  RotationArbitraryAxis=[0 0 1]  RotationSequenceAxes=FollowerAxes  RotationSequence=XYX  RotationSequenceAngles=[0 0 0]  RotationSequenceAnglesUnits=deg  RotationMatrix=[1 0 0;0 1 0;0 0 1]  Quaternion=[1 0 0 0]  TranslationMethod=None  TranslationCartesianOffset=[0 0 0]  TranslationCartesianOffsetUnits=m  TranslationStandardAxis=+Z  TranslationStandardOffset=0  TranslationStandardOffsetUnits=m  TranslationROffset=0  TranslationROffsetUnits=m  TranslationThetaOffset=0  TranslationThetaOffsetUnits=deg  TranslationZOffset=0  TranslationZOffsetUnits=m
  Idler roller ratio : Gain
  Idler roller solid : sm_lib/Body Elements/File Solid  ExtGeomFileName=CAD/roller_half_plain.step  UnitType=FromFile  ExtGeomFileUnits=m  StepReaderType=HEX  ExportConvexHullGeometry=off  InertiaType=CalculateFromGeometry  BasedOnType=Density  Density=convP.printDensity_kgm3  DensityUnits=kg/m^3  Mass=1  MassUnits=kg  CenterOfMass=[0 0 0]  CenterOfMassUnits=m  MomentsOfInertia=[1 1 1]  MomentsOfInertiaUnits=kg*m^2  ProductsOfInertia=[0 0 0]  ProductsOfInertiaUnits=kg*m^2  GraphicType=FromGeometry  MarkerShape=Sphere  MarkerSize=10  GraphicVisPropType=SimpleVisualProperties  GraphicDiffuseColor=[0.92 0.92 0.92]  GraphicOpacity=1  GraphicSpecularColor=[0.5 0.5 0.5 1.0]  GraphicAmbientColor=[0.15 0.15 0.15 1.0]  GraphicEmissiveColor=[0.0 0.0 0.0 1.0]  GraphicShininess=75  DoExposeReferenceFrame=on  SerializedFrames=<Frames/>
  Idler roller solid 2 : sm_lib/Body Elements/File Solid  ExtGeomFileName=CAD/roller_half_plain.step  UnitType=FromFile  ExtGeomFileUnits=m  StepReaderType=HEX  ExportConvexHullGeometry=off  InertiaType=CalculateFromGeometry  BasedOnType=Density  Density=convP.printDensity_kgm3  DensityUnits=kg/m^3  Mass=1  MassUnits=kg  CenterOfMass=[0 0 0]  CenterOfMassUnits=m  MomentsOfInertia=[1 1 1]  MomentsOfInertiaUnits=kg*m^2  ProductsOfInertia=[0 0 0]  ProductsOfInertiaUnits=kg*m^2  GraphicType=FromGeometry  MarkerShape=Sphere  MarkerSize=10  GraphicVisPropType=SimpleVisualProperties  GraphicDiffuseColor=[0.92 0.92 0.92]  GraphicOpacity=1  GraphicSpecularColor=[0.5 0.5 0.5 1.0]  GraphicAmbientColor=[0.15 0.15 0.15 1.0]  GraphicEmissiveColor=[0.0 0.0 0.0 1.0]  GraphicShininess=75  DoExposeReferenceFrame=on  SerializedFrames=<Frames/>
  Idler roller tooth phase : sm_lib/Frames and Transforms/Rigid Transform  RotationMethod=StandardAxis  FollAlignAxisA=+X  BaseAlignAxisA=+Y  FollAlignAxisB=+Y  BaseAlignAxisB=+Z  RotationStandardAxis=+Z  RotationAngle=0  RotationAngleUnits=deg  RotationArbitraryAxis=[0 0 1]  RotationSequenceAxes=FollowerAxes  RotationSequence=XYX  RotationSequenceAngles=[0 0 0]  RotationSequenceAnglesUnits=deg  RotationMatrix=[1 0 0;0 1 0;0 0 1]  Quaternion=[1 0 0 0]  TranslationMethod=None  TranslationCartesianOffset=[0 0 0]  TranslationCartesianOffsetUnits=m  TranslationStandardAxis=+Z  TranslationStandardOffset=0  TranslationStandardOffsetUnits=m  TranslationROffset=0  TranslationROffsetUnits=m  TranslationThetaOffset=0  TranslationThetaOffsetUnits=deg  TranslationZOffset=0  TranslationZOffsetUnits=m
  W : PMIOPort  Side=Left
  wires:
  drive roller angle (rad)/1 -> Idler roller ratio/1
  Idler roller ratio/1 -> Idler roller angle/1
  connections:
  W/RConn1 -- Idler roller axis/LConn1
  Idler roller axis/RConn1 -- Idler roller joint/LConn1
  Idler roller angle/RConn1 -- Idler roller joint/LConn2
  Idler roller joint/RConn1 -- Idler roller tooth phase/LConn1
  Idler roller solid/RConn1 -- Idler roller tooth phase/RConn1 -- Idler roller other half faces the other way/LConn1
  Idler roller other half faces the other way/RConn1 -- Idler roller solid 2/RConn1

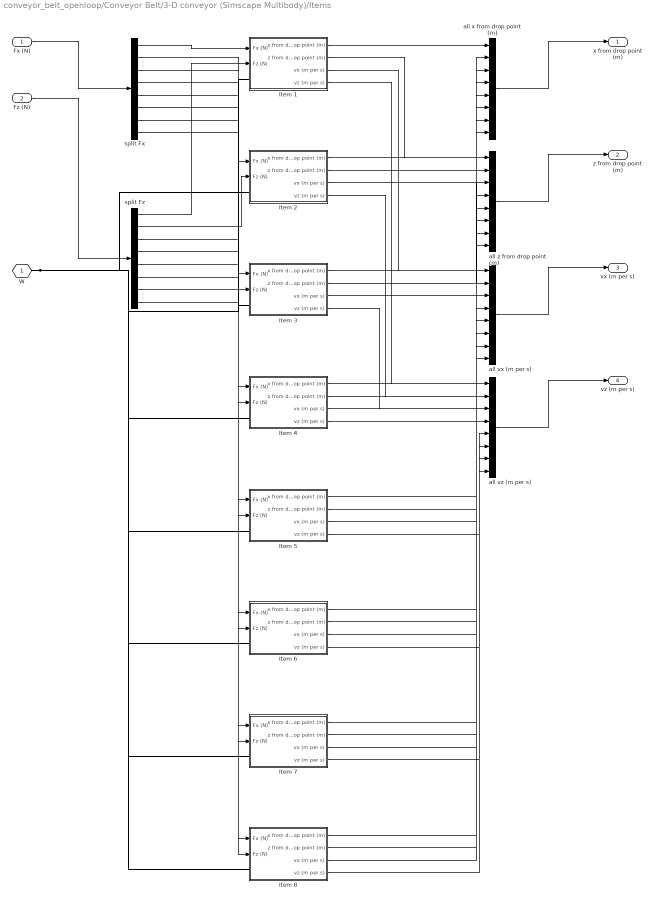
== system conveyor_belt_openloop/Conveyor Belt/3-D conveyor (Simscape Multibody)/Items ==
  Fx (N) : Inport
  Fz (N) : Inport  Port=2
  Item 1 : Subsystem
  Item 2 : Subsystem
  Item 3 : Subsystem
  Item 4 : Subsystem
  Item 5 : Subsystem
  Item 6 : Subsystem
  Item 7 : Subsystem
  Item 8 : Subsystem
  all vx (m per s) : Mux  Inputs=8
  all vz (m per s) : Mux  Inputs=8
  all x from drop point (m) : Mux  Inputs=8
  all z from drop point (m) : Mux  Inputs=8
  split Fx : Demux  Outputs=8
  split Fz : Demux  Outputs=8
  W : PMIOPort  Side=Left
  x from drop point (m) : Outport
  z from drop point (m) : Outport  Port=2
  vx (m per s) : Outport  Port=3
  vz (m per s) : Outport  Port=4
  wires:
  all x from drop point (m)/1 -> x from drop point (m)/1
  all z from drop point (m)/1 -> z from drop point (m)/1
  all vx (m per s)/1 -> vx (m per s)/1
  all vz (m per s)/1 -> vz (m per s)/1
  Fx (N)/1 -> split Fx/1
  Fz (N)/1 -> split Fz/1
  split Fx/1 -> Item 1/1(Fx (N))
  split Fz/1 -> Item 1/2(Fz (N))
  Item 1/1(x from drop point (m)) -> all x from drop point (m)/1
  Item 1/2(z from drop point (m)) -> all z from drop point (m)/1
  Item 1/3(vx (m per s)) -> all vx (m per s)/1
  Item 1/4(vz (m per s)) -> all vz (m per s)/1
  split Fx/2 -> Item 2/1(Fx (N))
  split Fz/2 -> Item 2/2(Fz (N))
  Item 2/1(x from drop point (m)) -> all x from drop point (m)/2
  Item 2/2(z from drop point (m)) -> all z from drop point (m)/2
  Item 2/3(vx (m per s)) -> all vx (m per s)/2
  Item 2/4(vz (m per s)) -> all vz (m per s)/2
  split Fx/3 -> Item 3/1(Fx (N))
  split Fz/3 -> Item 3/2(Fz (N))
  Item 3/1(x from drop point (m)) -> all x from drop point (m)/3
  Item 3/2(z from drop point (m)) -> all z from drop point (m)/3
  Item 3/3(vx (m per s)) -> all vx (m per s)/3
  Item 3/4(vz (m per s)) -> all vz (m per s)/3
  split Fx/4 -> Item 4/1(Fx (N))
  split Fz/4 -> Item 4/2(Fz (N))
  Item 4/1(x from drop point (m)) -> all x from drop point (m)/4
  Item 4/2(z from drop point (m)) -> all z from drop point (m)/4
  Item 4/3(vx (m per s)) -> all vx (m per s)/4
  Item 4/4(vz (m per s)) -> all vz (m per s)/4
  split Fx/5 -> Item 5/1(Fx (N))
  split Fz/5 -> Item 5/2(Fz (N))
  Item 5/1(x from drop point (m)) -> all x from drop point (m)/5
  Item 5/2(z from drop point (m)) -> all z from drop point (m)/5
  Item 5/3(vx (m per s)) -> all vx (m per s)/5
  Item 5/4(vz (m per s)) -> all vz (m per s)/5
  split Fx/6 -> Item 6/1(Fx (N))
  split Fz/6 -> Item 6/2(Fz (N))
  Item 6/1(x from drop point (m)) -> all x from drop point (m)/6
  Item 6/2(z from drop point (m)) -> all z from drop point (m)/6
  Item 6/3(vx (m per s)) -> all vx (m per s)/6
  Item 6/4(vz (m per s)) -> all vz (m per s)/6
  split Fx/7 -> Item 7/1(Fx (N))
  split Fz/7 -> Item 7/2(Fz (N))
  Item 7/1(x from drop point (m)) -> all x from drop point (m)/7
  Item 7/2(z from drop point (m)) -> all z from drop point (m)/7
  Item 7/3(vx (m per s)) -> all vx (m per s)/7
  Item 7/4(vz (m per s)) -> all vz (m per s)/7
  split Fx/8 -> Item 8/1(Fx (N))
  split Fz/8 -> Item 8/2(Fz (N))
  Item 8/1(x from drop point (m)) -> all x from drop point (m)/8
  Item 8/2(z from drop point (m)) -> all z from drop point (m)/8
  Item 8/3(vx (m per s)) -> all vx (m per s)/8
  Item 8/4(vz (m per s)) -> all vz (m per s)/8
  connections:
  Item 1/LConn1 -- W/RConn1 -- Item 2/LConn1 -- Item 3/LConn1 -- Item 4/LConn1 -- Item 5/LConn1 -- Item 6/LConn1 -- Item 7/LConn1 -- Item 8/LConn1
